simulink library "Transmission_Lib"  (R2025a)
settings: Solver=ode45  StartTime=0.0  StopTime=10.0  RelTol=1e-3  EnableMultiTasking=on
undefined symbols (not defined in the file): DCT_Param
libraries: fl_lib x45, nesl_utility x25, sdl_lib x18
(part 1 of 2)
Description:
  | Copyright 2014-2025 The MathWorks, Inc.
settings Model: Creator=smiller  LastModifiedBy=smiller
settings SolverCC: AlgebraicLoopSolver=TrustRegion
settings DataIOCC: SaveFormat=Array  SignalLoggingSaveFormat=ModelDataLogs  ReturnWorkspaceOutputs=off
settings OptimizationCC: ReuseModelBlockBuffer=off  ExpressionDepthLimit=2147483647.0  LifeSpan=inf
settings DebuggingCC: UnderspecifiedInitializationDetection=Classic  MergeDetectMultiDrivingBlocksExec=none  SolverPrmCheckMsg=warning  FcnCallInpInsideContextMsg=warning  UnconnectedInputMsg=warning  UnconnectedOutputMsg=warning  UnconnectedLineMsg=warning  AllowSymbolicDim=off  StateNameClashWarn=warning  PregeneratedLibrarySubsystemCodeDiagnostic=none  SFUnexpectedBacktrackingDiag=warning  SFNoUnconditionalDefaultTransitionDiag=warning  SFExecutionAtInitializationDiag=none  ArithmeticOperatorsInVariantConditions=warning
settings HardwareCC: ProdBitPerPointer=32.0  ProdBitPerSizeT=32.0  ProdBitPerPtrDiffT=32.0  ProdLargestAtomicFloat=None  ProdIntDivRoundTo=Undefined  ProdEndianess=Unspecified  ProdWordSize=32.0  ProdHWDeviceType=32-bit Generic
settings ModelReferenceCC: EnableRefExpFcnMdlSchedulingChecks=on  PropagateSignalLabelsOutOfModel=off
settings SFSimCC: SimUseLocalCustomCode=off  CustomCodeUndefinedFunction=UseInterfaceOnly
settings RTWCC: RTWUseLocalCustomCode=off  GPUComputeCapability=3.5  DLArmComputeVersion=19.05
settings CodeAppCC: StateflowObjectComments=on
settings GRTTargetCC: TargetLangStandard=C89/C90 (ANSI)  CombineOutputUpdateFcns=off  GRTInterface=on
settings ConfigComp: CovMetricSettings=dw  CovSaveCumulativeToWorkspaceVar=on  CovSaveSingleToWorkspaceVar=on  CovExternalEMLEnable=off  CovSFcnEnable=off

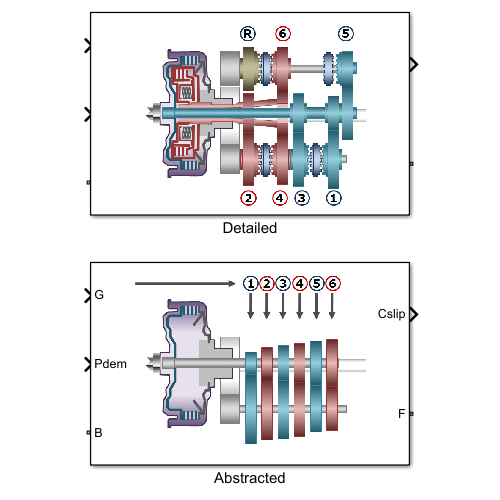
[thumbnail: Simulink's stored preview of the top-level diagram]
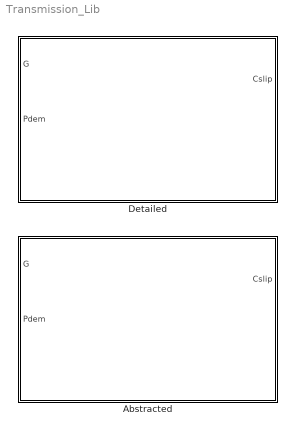
== system Transmission_Lib ==
  Abstracted : Subsystem
      mask Display: image(imread('DCT_Transmission_Abstracted_IMAGE2.jpg'));
  Detailed : Subsystem
      mask Display: image(imread('DCT_Transmission_IMAGE2.jpg'));

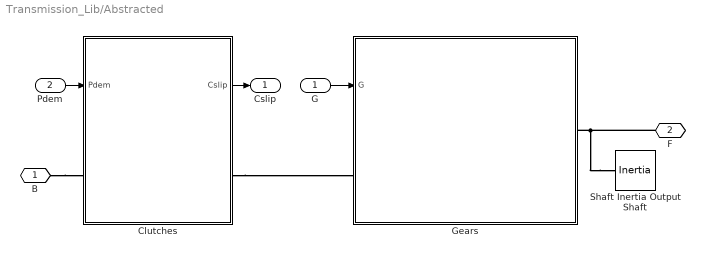
== system Transmission_Lib/Abstracted ==
  G : Inport
  Pdem : Inport  Port=2
  Clutches : Subsystem
      mask Display: image(imread('DCT_Clutches_Abstracted_IMAGE.jpg'));
  Gears : Subsystem
      mask Display: image(imread('DCT_Gears_Abstracted_IMAGE.jpg'));
  Shaft Inertia Output Shaft : fl_lib/Mechanical/Rotational Elements/Inertia  inertia=DCT_Param.Transmission.Shaft_Inertia_Output kg*m^2  num_ports=foundation.enum.numPorts2.one  w_specify=on  w_priority=High  w=DCT_Param.Transmission.Shaft_Velocity_Output rad/s  w_nominal_specify=off  w_nominal_value=1  w_nominal_unit=rad/s  t_specify=off  t_priority=High  t=0 N*m  t_nominal_specify=off  t_nominal_value=1  t_nominal_unit=N*m
  B : PMIOPort  Side=Left
  F : PMIOPort  Port=2  Side=Right
  Cslip : Outport  VectorParamsAs1DForOutWhenUnconnected=off
  wires:
  G/1 -> Gears/1(G)
  Clutches/1(Cslip) -> Cslip/1
  Pdem/1 -> Clutches/1(Pdem)
  connections:
  Shaft Inertia Output Shaft/LConn1 -- F/RConn1 -- Gears/RConn1
  Clutches/RConn1 -- Gears/LConn1
  B/RConn1 -- Clutches/LConn1

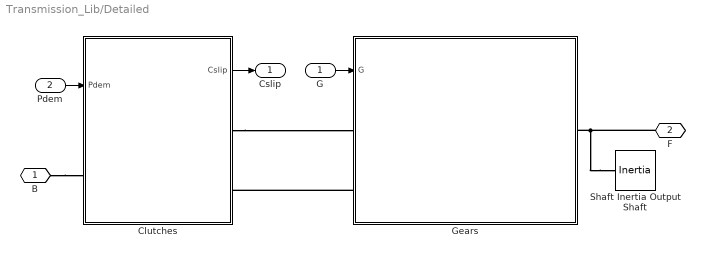
== system Transmission_Lib/Detailed ==
  G : Inport
  Pdem : Inport  Port=2
  Clutches : Subsystem
      mask Display:
      | image(imread('DCT_Clutches_IMAGE.jpg'));
      | port_label('input',1,'Pdem')
      | port_label('output',1,'Cslip')
      | port_label('LConn',1,'ICE')
      | port_label('RConn',1,'Odd')
      | port_label('RConn',2,'Even')
  Gears : Subsystem
      mask Display:
      | image(imread('DCT_Gears_IMAGE.jpg'));
      | port_label('input',1,'G')
      | port_label('LConn',1,'Odd')
      | port_label('LConn',2,'Even')
      | port_label('RConn',1,'F')
  Shaft Inertia Output Shaft : fl_lib/Mechanical/Rotational Elements/Inertia  inertia=DCT_Param.Transmission.Shaft_Inertia_Output kg*m^2  num_ports=foundation.enum.numPorts2.one  w_specify=on  w_priority=High  w=DCT_Param.Transmission.Shaft_Velocity_Output rad/s  w_nominal_specify=off  w_nominal_value=1  w_nominal_unit=rad/s  t_specify=off  t_priority=High  t=0 N*m  t_nominal_specify=off  t_nominal_value=1  t_nominal_unit=N*m
  B : PMIOPort  Side=Left
  F : PMIOPort  Port=2  Side=Right
  Cslip : Outport  VectorParamsAs1DForOutWhenUnconnected=off
  wires:
  G/1 -> Gears/1(G)
  Clutches/1(Cslip) -> Cslip/1
  Pdem/1 -> Clutches/1(Pdem)
  connections:
  Gears/LConn2 -- Clutches/RConn2
  Shaft Inertia Output Shaft/LConn1 -- F/RConn1 -- Gears/RConn1
  Clutches/RConn1 -- Gears/LConn1
  B/RConn1 -- Clutches/LConn1

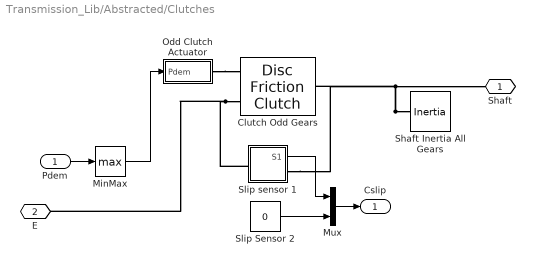
== system Transmission_Lib/Abstracted/Clutches ==
  Pdem : Inport
  Clutch Odd Gears : sdl_lib/Clutches/Disc Friction Clutch  geometry_model=1  r_eff=DCT_Param.Clutch.Torque_Radius mm  d_o=150 mm  d_i=100 mm  nS=DCT_Param.Clutch.Num_Friction_Surfaces  piston_area=DCT_Param.Clutch.Engagement_Piston_Area m^2  unidirectional=0  friction_model=1  mu_w_vector=[ 0 0.1 0.2 0.3 0.4 0.5 1 2 5 10 100 1000 ] rad/s  temperature_TLU=[280.0, 300.0, 320.0] K  mu_static=DCT_Param.Clutch.Static_Friction_Coeff  mu_static_vector=[0.4, 0.38, 0.36]  mu_coulomb=DCT_Param.Clutch.Kinetic_Friction_Coeff  mu_coulomb_vector=[ 0.29 0.28 0.26 0.22 0.21 0.2 0.2 0.19 0.19 0.19 0.19 0.19 ]  mu_coulomb_temp_vector=[0.3, 0.28, 0.25]  mu_coulomb_matrix=[0.34, 0.32, 0.3; 0.3, 0.28, 0.25; 0.25, 0.2, 0.15]  mu_interp_method=1  mu_extrap_method=1  d_f=DCT_Param.Clutch.Derating_Factor  w_tol=DCT_Param.Clutch.Clutch_Velocity_Tolerance rad/s  pressure_min=DCT_Param.Clutch.Threshold_Pressure Pa  mu_visc=DCT_Param.Clutch.Drag_Torque_Coeff N*m/(rad/s)  initial_state_locked=0  thermal_mass=25 kJ/K  T_init=300 K
      settings: InternalSimscapePortConfiguration="{\"Bottom\":[],\"Left\":[{\"id\":\"P\",\"label\":\"P\",\"type\":\"input\"},{\"id\":\"B\",\"label\":\"B\",\"type\":\"foundation.mechanical.rotational.rotational\"}],\"Right\":[{\"id\":\"F\",\"label\":\"F\",\"type\":\"foundation.mechanical.rotational.rotational\"}],\"Top\":[]}"
  MinMax : MinMax  Function=max
  Mux : Mux  Inputs=2
  Odd Clutch Actuator : Subsystem
  Shaft Inertia All Gears : fl_lib/Mechanical/Rotational Elements/Inertia  inertia=DCT_Param.Transmission.Shaft_Inertia_Odd kg*m^2  num_ports=foundation.enum.numPorts2.one  w_specify=on  w_priority=High  w=DCT_Param.Transmission.Shaft_Velocity_Odd rad/s  w_nominal_specify=off  w_nominal_value=1  w_nominal_unit=rad/s  t_specify=off  t_priority=High  t=0 N*m  t_nominal_specify=off  t_nominal_value=1  t_nominal_unit=N*m
  Slip Sensor 2 : Constant  Value=0
  Slip sensor 1 : Subsystem
  Shaft : PMIOPort  Side=Right
  E : PMIOPort  Port=2  Side=Left
  Cslip : Outport  VectorParamsAs1DForOutWhenUnconnected=off
  wires:
  Slip Sensor 2/1 -> Mux/2
  MinMax/1 -> Odd Clutch Actuator/1(Pdem)
  Pdem/1 -> MinMax/1
  Mux/1 -> Cslip/1
  Slip sensor 1/1(S1) -> Mux/1
  connections:
  Shaft Inertia All Gears/LConn1 -- Shaft/RConn1 -- Clutch Odd Gears/RConn1 -- Slip sensor 1/RConn1
  Odd Clutch Actuator/RConn1 -- Clutch Odd Gears/LConn1
  Clutch Odd Gears/LConn2 -- Slip sensor 1/LConn1 -- E/RConn1

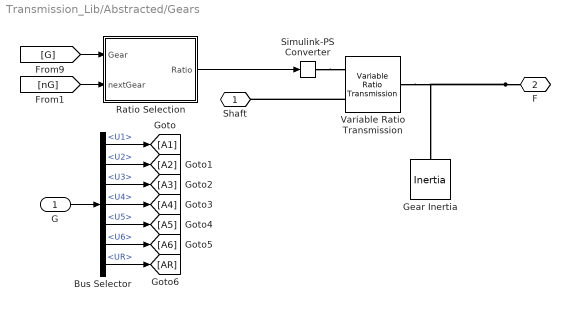
== system Transmission_Lib/Abstracted/Gears ==
  G : Inport
  Bus Selector : BusSelector  OutputSignals=U1,U2,U3,U4,U5,U6,UR
  Gear Inertia : fl_lib/Mechanical/Rotational Elements/Inertia  inertia=DCT_Param.Transmission.Gear_Inertia kg*m^2  num_ports=foundation.enum.numPorts2.one  w_specify=on  w_priority=High  w=0 rad/s  w_nominal_specify=off  w_nominal_value=1  w_nominal_unit=rad/s  t_specify=off  t_priority=High  t=0 N*m  t_nominal_specify=off  t_nominal_value=1  t_nominal_unit=N*m
  Ratio Selection : Subsystem
  Simulink-PS Converter : nesl_utility/Simulink-PS Converter  PhysicalDomain=network_engine_domain  SubClassName=ps_input  LeftPortType=input  RightPortType=output  PseudoPeriodic=off  Frequencies=[]  NoiseDistribution=none  NoiseParameters=[]  Unit=1  AffineConversion=off  FilteringAndDerivatives=zero  SimscapeFilterOrder=1  InputFilterTimeConstant=0.005  UdotUserProvided=0
  Variable Ratio Transmission : sdl_lib/Couplings & Drives/Variable Ratio Transmission  rotation_direction=3-2*(2)  kp=DCT_Param.Transmission.Abstract.Compliance N*m/rad  kv=DCT_Param.Transmission.Abstract.Damping N*m/(rad/s)  initial_torque=0 N*m  ratio_thr=0.01  losses_model=(1)-1  efficiency=0.85  pwr_thr=0.001 W  mu_visc=[ 0 0 ] N*m/(rad/s)
      settings: InternalSimscapePortConfiguration="{\"Bottom\":[],\"Left\":[{\"id\":\"ratio\",\"label\":\"r\",\"type\":\"input\"},{\"id\":\"B\",\"label\":\"B\",\"type\":\"foundation.mechanical.rotational.rotational\"}],\"Right\":[{\"id\":\"F\",\"label\":\"F\",\"type\":\"foundation.mechanical.rotational.rotational\"}],\"Top\":[]}"
  Shaft : PMIOPort  Side=Left
  F : PMIOPort  Port=2  Side=Right
  wires:
  [G] -> Ratio Selection/1(Gear)
  Ratio Selection/1(Ratio) -> Simulink-PS Converter/1
  Bus Selector/7 -> [AR]  "<UR>"
  Bus Selector/6 -> [A6]  "<U6>"
  Bus Selector/5 -> [A5]  "<U5>"
  Bus Selector/4 -> [A4]  "<U4>"
  Bus Selector/3 -> [A3]  "<U3>"
  Bus Selector/2 -> [A2]  "<U2>"
  Bus Selector/1 -> [A1]  "<U1>"
  G/1 -> Bus Selector/1
  [nG] -> Ratio Selection/2(nextGear)
  connections:
  Simulink-PS Converter/RConn1 -- Variable Ratio Transmission/LConn1
  F/RConn1 -- Gear Inertia/LConn1 -- Variable Ratio Transmission/RConn1
  Variable Ratio Transmission/LConn2 -- Shaft/RConn1

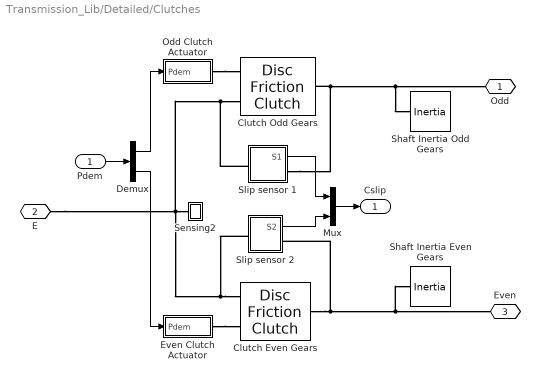
== system Transmission_Lib/Detailed/Clutches ==
  Pdem : Inport
  Clutch Even Gears : sdl_lib/Clutches/Disc Friction Clutch  Tag=CustomStyle  geometry_model=1  r_eff=DCT_Param.Clutch.Torque_Radius mm  d_o=150 mm  d_i=100 mm  nS=DCT_Param.Clutch.Num_Friction_Surfaces  piston_area=DCT_Param.Clutch.Engagement_Piston_Area m^2  unidirectional=0  friction_model=1  mu_w_vector=[ 0 0.1 0.2 0.3 0.4 0.5 1 2 5 10 100 1000 ] rad/s  temperature_TLU=[280.0, 300.0, 320.0] K  mu_static=DCT_Param.Clutch.Static_Friction_Coeff  mu_static_vector=[0.4, 0.38, 0.36]  mu_coulomb=DCT_Param.Clutch.Kinetic_Friction_Coeff  mu_coulomb_vector=[ 0.29 0.28 0.26 0.22 0.21 0.2 0.2 0.19 0.19 0.19 0.19 0.19 ]  mu_coulomb_temp_vector=[0.3, 0.28, 0.25]  mu_coulomb_matrix=[0.34, 0.32, 0.3; 0.3, 0.28, 0.25; 0.25, 0.2, 0.15]  mu_interp_method=1  mu_extrap_method=1  d_f=DCT_Param.Clutch.Derating_Factor  w_tol=DCT_Param.Clutch.Clutch_Velocity_Tolerance rad/s  pressure_min=DCT_Param.Clutch.Threshold_Pressure Pa  mu_visc=DCT_Param.Clutch.Drag_Torque_Coeff N*m/(rad/s)  initial_state_locked=0  thermal_mass=25 kJ/K  T_init=300 K
      settings: InternalSimscapePortConfiguration="{\"Bottom\":[],\"Left\":[{\"id\":\"P\",\"label\":\"P\",\"type\":\"input\"},{\"id\":\"B\",\"label\":\"B\",\"type\":\"foundation.mechanical.rotational.rotational\"}],\"Right\":[{\"id\":\"F\",\"label\":\"F\",\"type\":\"foundation.mechanical.rotational.rotational\"}],\"Top\":[]}"
  Clutch Odd Gears : sdl_lib/Clutches/Disc Friction Clutch  Tag=CustomStyle  geometry_model=1  r_eff=DCT_Param.Clutch.Torque_Radius mm  d_o=150 mm  d_i=100 mm  nS=DCT_Param.Clutch.Num_Friction_Surfaces  piston_area=DCT_Param.Clutch.Engagement_Piston_Area m^2  unidirectional=0  friction_model=1  mu_w_vector=[ 0 0.1 0.2 0.3 0.4 0.5 1 2 5 10 100 1000 ] rad/s  temperature_TLU=[280.0, 300.0, 320.0] K  mu_static=DCT_Param.Clutch.Static_Friction_Coeff  mu_static_vector=[0.4, 0.38, 0.36]  mu_coulomb=DCT_Param.Clutch.Kinetic_Friction_Coeff  mu_coulomb_vector=[ 0.29 0.28 0.26 0.22 0.21 0.2 0.2 0.19 0.19 0.19 0.19 0.19 ]  mu_coulomb_temp_vector=[0.3, 0.28, 0.25]  mu_coulomb_matrix=[0.34, 0.32, 0.3; 0.3, 0.28, 0.25; 0.25, 0.2, 0.15]  mu_interp_method=1  mu_extrap_method=1  d_f=DCT_Param.Clutch.Derating_Factor  w_tol=DCT_Param.Clutch.Clutch_Velocity_Tolerance rad/s  pressure_min=DCT_Param.Clutch.Threshold_Pressure Pa  mu_visc=DCT_Param.Clutch.Drag_Torque_Coeff N*m/(rad/s)  initial_state_locked=0  thermal_mass=25 kJ/K  T_init=300 K
      settings: InternalSimscapePortConfiguration="{\"Bottom\":[],\"Left\":[{\"id\":\"P\",\"label\":\"P\",\"type\":\"input\"},{\"id\":\"B\",\"label\":\"B\",\"type\":\"foundation.mechanical.rotational.rotational\"}],\"Right\":[{\"id\":\"F\",\"label\":\"F\",\"type\":\"foundation.mechanical.rotational.rotational\"}],\"Top\":[]}"
  Demux : Demux  Outputs=2
  Even Clutch Actuator : Subsystem
  Mux : Mux  Inputs=2
  Odd Clutch Actuator : Subsystem
  Sensing2 : Subsystem
  Shaft Inertia Even Gears : fl_lib/Mechanical/Rotational Elements/Inertia  inertia=DCT_Param.Transmission.Shaft_Inertia_Even kg*m^2  num_ports=foundation.enum.numPorts2.one  w_specify=on  w_priority=High  w=DCT_Param.Transmission.Shaft_Velocity_Even rad/s  w_nominal_specify=off  w_nominal_value=1  w_nominal_unit=rad/s  t_specify=off  t_priority=High  t=0 N*m  t_nominal_specify=off  t_nominal_value=1  t_nominal_unit=N*m
  Shaft Inertia Odd Gears : fl_lib/Mechanical/Rotational Elements/Inertia  inertia=DCT_Param.Transmission.Shaft_Inertia_Odd kg*m^2  num_ports=foundation.enum.numPorts2.one  w_specify=on  w_priority=High  w=DCT_Param.Transmission.Shaft_Velocity_Odd rad/s  w_nominal_specify=off  w_nominal_value=1  w_nominal_unit=rad/s  t_specify=off  t_priority=High  t=0 N*m  t_nominal_specify=off  t_nominal_value=1  t_nominal_unit=N*m
  Slip sensor 1 : Subsystem
  Slip sensor 2 : Subsystem
  Odd : PMIOPort  Side=Right
  E : PMIOPort  Port=2  Side=Left
  Even : PMIOPort  Port=3  Side=Right
  Cslip : Outport  VectorParamsAs1DForOutWhenUnconnected=off
  wires:
  Demux/2 -> Even Clutch Actuator/1(Pdem)
  Demux/1 -> Odd Clutch Actuator/1(Pdem)
  Pdem/1 -> Demux/1
  Mux/1 -> Cslip/1
  Slip sensor 2/1(S2) -> Mux/2
  Slip sensor 1/1(S1) -> Mux/1
  connections:
  Shaft Inertia Odd Gears/LConn1 -- Odd/RConn1 -- Clutch Odd Gears/RConn1 -- Slip sensor 1/RConn1
  Odd Clutch Actuator/RConn1 -- Clutch Odd Gears/LConn1
  Shaft Inertia Even Gears/LConn1 -- Even/RConn1 -- Clutch Even Gears/RConn1 -- Slip sensor 2/RConn1
  Clutch Even Gears/LConn2 -- Slip sensor 2/LConn1 -- E/RConn1 -- Sensing2/LConn1 -- Clutch Odd Gears/LConn2 -- Slip sensor 1/LConn1
  Even Clutch Actuator/RConn1 -- Clutch Even Gears/LConn1

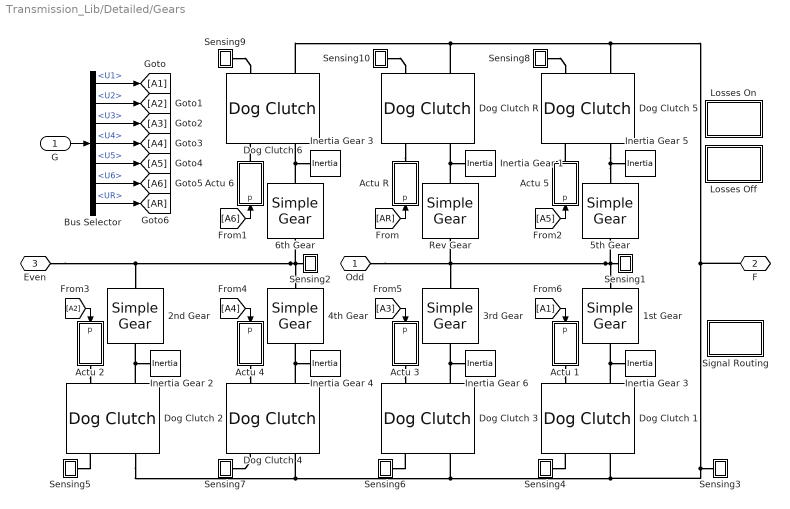
== system Transmission_Lib/Detailed/Gears ==
  G : Inport
  1st Gear : sdl_lib/Gears/Simple Gear  Tag=CustomStyle  ratio=DCT_Param.Transmission.Ratios(1)  rotation_direction=3-2*(2)  friction_model=1  T_noload=0.1 N*m  T_nom=5 N*m  efficiency_nom=0.8  efficiency=DCT_Param.Transmission.Gear_Efficiency  temperature_TLU=[ 280 300 320 ] K  load_TLU=[ 1 5 10 ] N*m  efficiency_TLU=[ 0.95 0.9 0.85 ]  efficiency_TLU2=[ 0.85 0.8 0.75; 0.95 0.9 0.85; 0.85 0.8 0.7 ]  w_thr=DCT_Param.Transmission.Gear_Ang_Vel_Thr rad/s  pwr_thr=0.001 W  enable_backlash=false  hardstop_model=simscape.enum.hardstop.smooth  backlash_distance=1e-3 mm  r_base=0.1 m  transition=1e-4 mm  backlash_stiffness=1e7 N/m  backlash_damping=1e6 N*s/m  coeff_rest=0  v_tol=0.001 m/s  f_tol=0 N  mu_visc=[0 0] N*m/(rad/s)  thermal_mass=50 J/K  temperature_specify=off  temperature_priority=High  temperature=300 K  temperature_nominal_specify=off  temperature_nominal_value=1  temperature_nominal_unit=K  x_backlash_specify=off  x_backlash_priority=None  x_backlash=0 mm  x_backlash_nominal_specify=off  x_backlash_nominal_value=1  x_backlash_nominal_unit=mm  f_hardstop_specify=off  f_hardstop_priority=None  f_hardstop=0 N  f_hardstop_nominal_specify=off  f_hardstop_nominal_value=1  f_hardstop_nominal_unit=N  v_backlash_specify=off  v_backlash_priority=None  v_backlash=0 m/s  v_backlash_nominal_specify=off  v_backlash_nominal_value=1  v_backlash_nominal_unit=m/s
  2nd Gear : sdl_lib/Gears/Simple Gear  Tag=CustomStyle  ratio=DCT_Param.Transmission.Ratios(2)  rotation_direction=3-2*(2)  friction_model=1  T_noload=0.1 N*m  T_nom=5 N*m  efficiency_nom=0.8  efficiency=DCT_Param.Transmission.Gear_Efficiency  temperature_TLU=[ 280 300 320 ] K  load_TLU=[ 1 5 10 ] N*m  efficiency_TLU=[ 0.95 0.9 0.85 ]  efficiency_TLU2=[ 0.85 0.8 0.75; 0.95 0.9 0.85; 0.85 0.8 0.7 ]  w_thr=DCT_Param.Transmission.Gear_Ang_Vel_Thr rad/s  pwr_thr=0.001 W  enable_backlash=false  hardstop_model=simscape.enum.hardstop.smooth  backlash_distance=1e-3 mm  r_base=0.1 m  transition=1e-4 mm  backlash_stiffness=1e7 N/m  backlash_damping=1e6 N*s/m  coeff_rest=0  v_tol=0.001 m/s  f_tol=0 N  mu_visc=[0 0] N*m/(rad/s)  thermal_mass=50 J/K  temperature_specify=off  temperature_priority=High  temperature=300 K  temperature_nominal_specify=off  temperature_nominal_value=1  temperature_nominal_unit=K  x_backlash_specify=off  x_backlash_priority=None  x_backlash=0 mm  x_backlash_nominal_specify=off  x_backlash_nominal_value=1  x_backlash_nominal_unit=mm  f_hardstop_specify=off  f_hardstop_priority=None  f_hardstop=0 N  f_hardstop_nominal_specify=off  f_hardstop_nominal_value=1  f_hardstop_nominal_unit=N  v_backlash_specify=off  v_backlash_priority=None  v_backlash=0 m/s  v_backlash_nominal_specify=off  v_backlash_nominal_value=1  v_backlash_nominal_unit=m/s
  3rd Gear : sdl_lib/Gears/Simple Gear  Tag=CustomStyle  ratio=DCT_Param.Transmission.Ratios(3)  rotation_direction=3-2*(2)  friction_model=1  T_noload=0.1 N*m  T_nom=5 N*m  efficiency_nom=0.8  efficiency=DCT_Param.Transmission.Gear_Efficiency  temperature_TLU=[ 280 300 320 ] K  load_TLU=[ 1 5 10 ] N*m  efficiency_TLU=[ 0.95 0.9 0.85 ]  efficiency_TLU2=[ 0.85 0.8 0.75; 0.95 0.9 0.85; 0.85 0.8 0.7 ]  w_thr=DCT_Param.Transmission.Gear_Ang_Vel_Thr rad/s  pwr_thr=0.001 W  enable_backlash=false  hardstop_model=simscape.enum.hardstop.smooth  backlash_distance=1e-3 mm  r_base=0.1 m  transition=1e-4 mm  backlash_stiffness=1e7 N/m  backlash_damping=1e6 N*s/m  coeff_rest=0  v_tol=0.001 m/s  f_tol=0 N  mu_visc=[0 0] N*m/(rad/s)  thermal_mass=50 J/K  temperature_specify=off  temperature_priority=High  temperature=300 K  temperature_nominal_specify=off  temperature_nominal_value=1  temperature_nominal_unit=K  x_backlash_specify=off  x_backlash_priority=None  x_backlash=0 mm  x_backlash_nominal_specify=off  x_backlash_nominal_value=1  x_backlash_nominal_unit=mm  f_hardstop_specify=off  f_hardstop_priority=None  f_hardstop=0 N  f_hardstop_nominal_specify=off  f_hardstop_nominal_value=1  f_hardstop_nominal_unit=N  v_backlash_specify=off  v_backlash_priority=None  v_backlash=0 m/s  v_backlash_nominal_specify=off  v_backlash_nominal_value=1  v_backlash_nominal_unit=m/s
  4th Gear : sdl_lib/Gears/Simple Gear  Tag=CustomStyle  ratio=DCT_Param.Transmission.Ratios(4)  rotation_direction=3-2*(2)  friction_model=1  T_noload=0.1 N*m  T_nom=5 N*m  efficiency_nom=0.8  efficiency=DCT_Param.Transmission.Gear_Efficiency  temperature_TLU=[ 280 300 320 ] K  load_TLU=[ 1 5 10 ] N*m  efficiency_TLU=[ 0.95 0.9 0.85 ]  efficiency_TLU2=[ 0.85 0.8 0.75; 0.95 0.9 0.85; 0.85 0.8 0.7 ]  w_thr=DCT_Param.Transmission.Gear_Ang_Vel_Thr rad/s  pwr_thr=0.001 W  enable_backlash=false  hardstop_model=simscape.enum.hardstop.smooth  backlash_distance=1e-3 mm  r_base=0.1 m  transition=1e-4 mm  backlash_stiffness=1e7 N/m  backlash_damping=1e6 N*s/m  coeff_rest=0  v_tol=0.001 m/s  f_tol=0 N  mu_visc=[0 0] N*m/(rad/s)  thermal_mass=50 J/K  temperature_specify=off  temperature_priority=High  temperature=300 K  temperature_nominal_specify=off  temperature_nominal_value=1  temperature_nominal_unit=K  x_backlash_specify=off  x_backlash_priority=None  x_backlash=0 mm  x_backlash_nominal_specify=off  x_backlash_nominal_value=1  x_backlash_nominal_unit=mm  f_hardstop_specify=off  f_hardstop_priority=None  f_hardstop=0 N  f_hardstop_nominal_specify=off  f_hardstop_nominal_value=1  f_hardstop_nominal_unit=N  v_backlash_specify=off  v_backlash_priority=None  v_backlash=0 m/s  v_backlash_nominal_specify=off  v_backlash_nominal_value=1  v_backlash_nominal_unit=m/s
  5th Gear : sdl_lib/Gears/Simple Gear  Tag=CustomStyle  ratio=DCT_Param.Transmission.Ratios(5)  rotation_direction=3-2*(2)  friction_model=1  T_noload=0.1 N*m  T_nom=5 N*m  efficiency_nom=0.8  efficiency=DCT_Param.Transmission.Gear_Efficiency  temperature_TLU=[ 280 300 320 ] K  load_TLU=[ 1 5 10 ] N*m  efficiency_TLU=[ 0.95 0.9 0.85 ]  efficiency_TLU2=[ 0.85 0.8 0.75; 0.95 0.9 0.85; 0.85 0.8 0.7 ]  w_thr=DCT_Param.Transmission.Gear_Ang_Vel_Thr rad/s  pwr_thr=0.001 W  enable_backlash=false  hardstop_model=simscape.enum.hardstop.smooth  backlash_distance=1e-3 mm  r_base=0.1 m  transition=1e-4 mm  backlash_stiffness=1e7 N/m  backlash_damping=1e6 N*s/m  coeff_rest=0  v_tol=0.001 m/s  f_tol=0 N  mu_visc=[0 0] N*m/(rad/s)  thermal_mass=50 J/K  temperature_specify=off  temperature_priority=High  temperature=300 K  temperature_nominal_specify=off  temperature_nominal_value=1  temperature_nominal_unit=K  x_backlash_specify=off  x_backlash_priority=None  x_backlash=0 mm  x_backlash_nominal_specify=off  x_backlash_nominal_value=1  x_backlash_nominal_unit=mm  f_hardstop_specify=off  f_hardstop_priority=None  f_hardstop=0 N  f_hardstop_nominal_specify=off  f_hardstop_nominal_value=1  f_hardstop_nominal_unit=N  v_backlash_specify=off  v_backlash_priority=None  v_backlash=0 m/s  v_backlash_nominal_specify=off  v_backlash_nominal_value=1  v_backlash_nominal_unit=m/s
  6th Gear : sdl_lib/Gears/Simple Gear  Tag=CustomStyle  ratio=DCT_Param.Transmission.Ratios(6)  rotation_direction=3-2*(2)  friction_model=1  T_noload=0.1 N*m  T_nom=5 N*m  efficiency_nom=0.8  efficiency=DCT_Param.Transmission.Gear_Efficiency  temperature_TLU=[ 280 300 320 ] K  load_TLU=[ 1 5 10 ] N*m  efficiency_TLU=[ 0.95 0.9 0.85 ]  efficiency_TLU2=[ 0.85 0.8 0.75; 0.95 0.9 0.85; 0.85 0.8 0.7 ]  w_thr=DCT_Param.Transmission.Gear_Ang_Vel_Thr rad/s  pwr_thr=0.001 W  enable_backlash=false  hardstop_model=simscape.enum.hardstop.smooth  backlash_distance=1e-3 mm  r_base=0.1 m  transition=1e-4 mm  backlash_stiffness=1e7 N/m  backlash_damping=1e6 N*s/m  coeff_rest=0  v_tol=0.001 m/s  f_tol=0 N  mu_visc=[0 0] N*m/(rad/s)  thermal_mass=50 J/K  temperature_specify=off  temperature_priority=High  temperature=300 K  temperature_nominal_specify=off  temperature_nominal_value=1  temperature_nominal_unit=K  x_backlash_specify=off  x_backlash_priority=None  x_backlash=0 mm  x_backlash_nominal_specify=off  x_backlash_nominal_value=1  x_backlash_nominal_unit=mm  f_hardstop_specify=off  f_hardstop_priority=None  f_hardstop=0 N  f_hardstop_nominal_specify=off  f_hardstop_nominal_value=1  f_hardstop_nominal_unit=N  v_backlash_specify=off  v_backlash_priority=None  v_backlash=0 m/s  v_backlash_nominal_specify=off  v_backlash_nominal_value=1  v_backlash_nominal_unit=m/s
  Actu 1 : Subsystem
  Actu 2 : Subsystem
  Actu 3 : Subsystem
  Actu 4 : Subsystem
  Actu 5 : Subsystem
  Actu 6 : Subsystem
  Actu R : Subsystem
  Bus Selector : BusSelector  OutputSignals=U1,U2,U3,U4,U5,U6,UR
  Dog Clutch 1 : sdl_lib/Clutches/Dog Clutch  Tag=CustomStyle  model=1  w_threshold=5 rpm  thermal_port=simscape.enum.thermaleffects.omit  radius=DCT_Param.Dog_Clutch.Teeth_Mean_Radius mm  max_torque=DCT_Param.Dog_Clutch.Max_Torque N*m  n_teeth=6  temperature_TLU=[280.0, 300.0, 320.0] K  max_torque_vector=[1000.0, 1050.0, 1000.0] N*m  interp_method=1  extrap_method=1  clutch_backlash=10 deg  clutch_stiffness=1e+7 N*m/rad  clutch_damping=2 N*m/(rad/s)  shift_linkage_twomode=sdl.enum.shift_linkage_twomode.logic  shift_linkage=sdl.enum.shift_linkage.conserving  tooth_height=DCT_Param.Dog_Clutch.Tooth_Height mm  ring_hub_gap=DCT_Param.Dog_Clutch.Ring_Hub_Clearance mm  back_stop=1  transl_stiffness=DCT_Param.Dog_Clutch.Ring_Stop_Stiffness N/m  transl_damping=DCT_Param.Dog_Clutch.Ring_Stop_Damping N/(m/s)  visc_fric_transl=DCT_Param.Dog_Clutch.Shift_Linkage_Damping N/(m/s)  engaged_fric_transl=100 N*s/m  disengaged_fric_transl=50 N*s/m  v_tol=0.1 m/s  f_tol=0.001 N  fric_coeff=0.05  direction=3-2*(1)  engagement_velocity=DCT_Param.Dog_Clutch.Max_Engage_Velocity rad/s  engagement_overlap=DCT_Param.Dog_Clutch.Tooth_Engage_Overlap mm  engagement_block_stiffness=10e6 N/m  engagement_block_damping=300 N*s/m  initial_state_engaged=1  init_pos=DCT_Param.Dog_Clutch.Tooth_Height+DCT_Param.Dog_Clutch.Ring_Hub_Clearance mm  init_rel_angle=0 deg  thermal_mass=25 kJ/K  T_init=300 K
      settings: InternalSimscapePortConfiguration="{\"Bottom\":[],\"Left\":[{\"id\":\"S\",\"label\":\"S\",\"type\":\"foundation.mechanical.translational.translational\"},{\"id\":\"R\",\"label\":\"R\",\"type\":\"foundation.mechanical.rotational.rotational\"}],\"Right\":[{\"id\":\"X\",\"label\":\"X\",\"type\":\"output\"},{\"id\":\"H\",\"label\":\"H\",\"type\":\"foundation.mechanical.rotational.rotational\"}],\"Top\":[]}"
  Dog Clutch {2..6} (5 alike) : sdl_lib/Clutches/Dog Clutch  Tag=CustomStyle  model=1  w_threshold=5 rpm  thermal_port=simscape.enum.thermaleffects.omit  radius=DCT_Param.Dog_Clutch.Teeth_Mean_Radius mm  max_torque=DCT_Param.Dog_Clutch.Max_Torque N*m  n_teeth=6  temperature_TLU=[280.0, 300.0, 320.0] K  max_torque_vector=[1000.0, 1050.0, 1000.0] N*m  interp_method=1  extrap_method=1  clutch_backlash=10 deg  clutch_stiffness=1e+7 N*m/rad  clutch_damping=2 N*m/(rad/s)  shift_linkage_twomode=sdl.enum.shift_linkage_twomode.logic  shift_linkage=sdl.enum.shift_linkage.conserving  tooth_height=DCT_Param.Dog_Clutch.Tooth_Height mm  ring_hub_gap=DCT_Param.Dog_Clutch.Ring_Hub_Clearance mm  back_stop=1  transl_stiffness=DCT_Param.Dog_Clutch.Ring_Stop_Stiffness N/m  transl_damping=DCT_Param.Dog_Clutch.Ring_Stop_Damping N/(m/s)  visc_fric_transl=DCT_Param.Dog_Clutch.Shift_Linkage_Damping N/(m/s)  engaged_fric_transl=100 N*s/m  disengaged_fric_transl=50 N*s/m  v_tol=0.1 m/s  f_tol=0.001 N  fric_coeff=0.05  direction=3-2*(1)  engagement_velocity=DCT_Param.Dog_Clutch.Max_Engage_Velocity rad/s  engagement_overlap=DCT_Param.Dog_Clutch.Tooth_Engage_Overlap mm  engagement_block_stiffness=10e6 N/m  engagement_block_damping=300 N*s/m  initial_state_engaged=0  init_pos=0 mm  init_rel_angle=0 deg  thermal_mass=25 kJ/K  T_init=300 K
      settings: InternalSimscapePortConfiguration="{\"Bottom\":[],\"Left\":[{\"id\":\"S\",\"label\":\"S\",\"type\":\"foundation.mechanical.translational.translational\"},{\"id\":\"R\",\"label\":\"R\",\"type\":\"foundation.mechanical.rotational.rotational\"}],\"Right\":[{\"id\":\"X\",\"label\":\"X\",\"type\":\"output\"},{\"id\":\"H\",\"label\":\"H\",\"type\":\"foundation.mechanical.rotational.rotational\"}],\"Top\":[]}"
  Dog Clutch R : sdl_lib/Clutches/Dog Clutch  Tag=CustomStyle  model=1  w_threshold=5 rpm  thermal_port=simscape.enum.thermaleffects.omit  radius=DCT_Param.Dog_Clutch.Teeth_Mean_Radius mm  max_torque=DCT_Param.Dog_Clutch.Max_Torque N*m  n_teeth=6  temperature_TLU=[280.0, 300.0, 320.0] K  max_torque_vector=[1000.0, 1050.0, 1000.0] N*m  interp_method=1  extrap_method=1  clutch_backlash=10 deg  clutch_stiffness=1e+7 N*m/rad  clutch_damping=2 N*m/(rad/s)  shift_linkage_twomode=sdl.enum.shift_linkage_twomode.logic  shift_linkage=sdl.enum.shift_linkage.conserving  tooth_height=DCT_Param.Dog_Clutch.Tooth_Height mm  ring_hub_gap=DCT_Param.Dog_Clutch.Ring_Hub_Clearance mm  back_stop=1  transl_stiffness=DCT_Param.Dog_Clutch.Ring_Stop_Stiffness N/m  transl_damping=DCT_Param.Dog_Clutch.Ring_Stop_Damping N/(m/s)  visc_fric_transl=DCT_Param.Dog_Clutch.Shift_Linkage_Damping N/(m/s)  engaged_fric_transl=100 N*s/m  disengaged_fric_transl=50 N*s/m  v_tol=0.1 m/s  f_tol=0.001 N  fric_coeff=0.05  direction=3-2*(1)  engagement_velocity=DCT_Param.Dog_Clutch.Max_Engage_Velocity rad/s  engagement_overlap=DCT_Param.Dog_Clutch.Tooth_Engage_Overlap mm  engagement_block_stiffness=10e6 N/m  engagement_block_damping=300 N*s/m  initial_state_engaged=0  init_pos=0 mm  init_rel_angle=0 deg  thermal_mass=25 kJ/K  T_init=300 K
      settings: InternalSimscapePortConfiguration="{\"Bottom\":[],\"Left\":[{\"id\":\"S\",\"label\":\"S\",\"type\":\"foundation.mechanical.translational.translational\"},{\"id\":\"R\",\"label\":\"R\",\"type\":\"foundation.mechanical.rotational.rotational\"}],\"Right\":[{\"id\":\"X\",\"label\":\"X\",\"type\":\"output\"},{\"id\":\"H\",\"label\":\"H\",\"type\":\"foundation.mechanical.rotational.rotational\"}],\"Top\":[]}"
  Inertia Gear {1..6} (6 alike) : fl_lib/Mechanical/Rotational Elements/Inertia  inertia=DCT_Param.Transmission.Gear_Inertia kg*m^2  num_ports=foundation.enum.numPorts2.one  w_specify=on  w_priority=High  w=DCT_Param.Transmission.Gear_Initial_Velocity rad/s  w_nominal_specify=off  w_nominal_value=1  w_nominal_unit=rad/s  t_specify=off  t_priority=High  t=0 N*m  t_nominal_specify=off  t_nominal_value=1  t_nominal_unit=N*m
  "Inertia Gear 3 " : fl_lib/Mechanical/Rotational Elements/Inertia  inertia=DCT_Param.Transmission.Gear_Inertia kg*m^2  num_ports=foundation.enum.numPorts2.one  w_specify=on  w_priority=High  w=DCT_Param.Transmission.Gear_Initial_Velocity rad/s  w_nominal_specify=off  w_nominal_value=1  w_nominal_unit=rad/s  t_specify=off  t_priority=High  t=0 N*m  t_nominal_specify=off  t_nominal_value=1  t_nominal_unit=N*m
  Losses Off : Subsystem
      settings: OpenFcn=|
      | gearblk_h = find_system(gcs,'MatchFilter',@Simulink.match.allVariants,'ClassName','simple_gear');
      | for i = 1:length(gearblk_h)
      | set_param(gearblk_h{i},'friction_model','1'); end
      mask Display: disp('Losses\nOff');
  Losses On : Subsystem
      settings: OpenFcn=|
      | gearblk_h = find_system(gcs,'MatchFilter',@Simulink.match.allVariants,'ClassName','simple_gear');
      | for i = 1:length(gearblk_h)
      | set_param(gearblk_h{i},'friction_model','2'); end;
      mask Display: disp('Losses\nOn');
  Rev Gear : sdl_lib/Gears/Simple Gear  Tag=CustomStyle  ratio=DCT_Param.Transmission.Ratios(1)  rotation_direction=3-2*(1)  friction_model=1  T_noload=0.1 N*m  T_nom=5 N*m  efficiency_nom=0.8  efficiency=DCT_Param.Transmission.Gear_Efficiency  temperature_TLU=[ 280 300 320 ] K  load_TLU=[ 1 5 10 ] N*m  efficiency_TLU=[ 0.95 0.9 0.85 ]  efficiency_TLU2=[ 0.85 0.8 0.75; 0.95 0.9 0.85; 0.85 0.8 0.7 ]  w_thr=DCT_Param.Transmission.Gear_Ang_Vel_Thr rad/s  pwr_thr=0.001 W  enable_backlash=false  hardstop_model=simscape.enum.hardstop.smooth  backlash_distance=1e-3 mm  r_base=0.1 m  transition=1e-4 mm  backlash_stiffness=1e7 N/m  backlash_damping=1e6 N*s/m  coeff_rest=0  v_tol=0.001 m/s  f_tol=0 N  mu_visc=[0 0] N*m/(rad/s)  thermal_mass=50 J/K  temperature_specify=off  temperature_priority=High  temperature=300 K  temperature_nominal_specify=off  temperature_nominal_value=1  temperature_nominal_unit=K  x_backlash_specify=off  x_backlash_priority=None  x_backlash=0 mm  x_backlash_nominal_specify=off  x_backlash_nominal_value=1  x_backlash_nominal_unit=mm  f_hardstop_specify=off  f_hardstop_priority=None  f_hardstop=0 N  f_hardstop_nominal_specify=off  f_hardstop_nominal_value=1  f_hardstop_nominal_unit=N  v_backlash_specify=off  v_backlash_priority=None  v_backlash=0 m/s  v_backlash_nominal_specify=off  v_backlash_nominal_value=1  v_backlash_nominal_unit=m/s
  Sensing1 : Subsystem
  Sensing10 : Subsystem
  Sensing2 : Subsystem
  Sensing3 : Subsystem
  Sensing4 : Subsystem
  Sensing5 : Subsystem
  Sensing6 : Subsystem
  Sensing7 : Subsystem
  Sensing8 : Subsystem
  Sensing9 : Subsystem
  Signal Routing : Subsystem
  Odd : PMIOPort  Side=Left
  F : PMIOPort  Port=2  Side=Right
  Even : PMIOPort  Port=3  Side=Left
  wires:
  Bus Selector/7 -> [AR]  "<UR>"
  [AR] -> Actu R/1(p)
  [A1] -> Actu 1/1(p)
  Bus Selector/6 -> [A6]  "<U6>"
  Bus Selector/5 -> [A5]  "<U5>"
  Bus Selector/4 -> [A4]  "<U4>"
  Bus Selector/3 -> [A3]  "<U3>"
  Bus Selector/2 -> [A2]  "<U2>"
  Bus Selector/1 -> [A1]  "<U1>"
  [A3] -> Actu 3/1(p)
  [A4] -> Actu 4/1(p)
  [A2] -> Actu 2/1(p)
  [A5] -> Actu 5/1(p)
  [A6] -> Actu 6/1(p)
  G/1 -> Bus Selector/1
  connections:
  Sensing10/LConn1 -- Dog Clutch R/RConn1
  Sensing9/LConn1 -- Dog Clutch 6/RConn1
  Sensing8/LConn1 -- Dog Clutch 5/RConn1
  Sensing7/LConn1 -- Dog Clutch 4/RConn1
  Sensing6/LConn1 -- Dog Clutch 3/RConn1
  Sensing5/LConn1 -- Dog Clutch 2/RConn1
  Sensing4/LConn1 -- Dog Clutch 1/RConn1
  Dog Clutch R/LConn1 -- Actu R/RConn1
  Dog Clutch R/LConn2 -- Rev Gear/RConn1 -- Inertia Gear 1/LConn1
  Sensing3/LConn1 -- Dog Clutch 1/RConn2 -- Dog Clutch 3/RConn2 -- Dog Clutch 4/RConn2 -- Dog Clutch 2/RConn2 -- F/RConn1 -- Dog Clutch 5/RConn2 -- Dog Clutch R/RConn2 -- Dog Clutch 6/RConn2
  5th Gear/LConn1 -- Rev Gear/LConn1 -- 3rd Gear/LConn1 -- Odd/RConn1 -- Sensing1/LConn1 -- 1st Gear/LConn1
  6th Gear/LConn1 -- 2nd Gear/LConn1 -- Even/RConn1 -- Sensing2/LConn1 -- 4th Gear/LConn1
  Actu 1/RConn1 -- Dog Clutch 1/LConn1
  Dog Clutch 1/LConn2 -- 1st Gear/RConn1 -- Inertia Gear 3/LConn1
  Actu 4/RConn1 -- Dog Clutch 4/LConn1
  Actu 5/RConn1 -- Dog Clutch 5/LConn1
  Actu 6/RConn1 -- Dog Clutch 6/LConn1
  Actu 2/RConn1 -- Dog Clutch 2/LConn1
  Actu 3/RConn1 -- Dog Clutch 3/LConn1
  3rd Gear/RConn1 -- Dog Clutch 3/LConn2 -- Inertia Gear 6/LConn1
  4th Gear/RConn1 -- Dog Clutch 4/LConn2 -- Inertia Gear 4/LConn1
  2nd Gear/RConn1 -- Dog Clutch 2/LConn2 -- Inertia Gear 2/LConn1
  5th Gear/RConn1 -- Dog Clutch 5/LConn2 -- Inertia Gear 5/LConn1
  Dog Clutch 6/LConn2 -- 6th Gear/RConn1 -- "Inertia Gear 3 "/LConn1

== system Transmission_Lib/Abstracted/Clutches/Odd Clutch Actuator ==
  Pdem : Inport
  Pressure controller time constant : TransferFcn  Denominator=[0.02 1]
  Simulink-PS Converter : nesl_utility/Simulink-PS Converter  PhysicalDomain=network_engine_domain  SubClassName=ps_input  LeftPortType=input  RightPortType=output  PseudoPeriodic=off  Frequencies=[]  NoiseDistribution=none  NoiseParameters=[]  Unit=Pa  AffineConversion=off  FilteringAndDerivatives=zero  SimscapeFilterOrder=1  InputFilterTimeConstant=0.005  UdotUserProvided=0
  P : PMIOPort  Side=Right
  wires:
  Pdem/1 -> Pressure controller time constant/1
  Pressure controller time constant/1 -> Simulink-PS Converter/1
  connections:
  P/RConn1 -- Simulink-PS Converter/RConn1

== system Transmission_Lib/Abstracted/Clutches/Slip sensor 1 ==
  Ideal Rotational Motion Sensor : fl_lib/Mechanical/Mechanical Sensors/Ideal Rotational Motion Sensor  reference=foundation.enum.MeasurementReference.difference  acceleration_port=false  velocity_port=true  position_port=true  wrap_angle=simscape.enum.onoff.off  offset=0 rad
  PS-Simulink Converter3 : nesl_utility/PS-Simulink Converter  PhysicalDomain=network_engine_domain  SubClassName=ps_output  LeftPortType=input  RightPortType=output  PseudoPeriodic=off  Frequencies=[]  VectorFormat=1-D array  Unit=rpm  AffineConversion=off
  Zero-Order Hold : ZeroOrderHold  SampleTime=0.01
  F : PMIOPort  Side=Right
  B : PMIOPort  Port=2  Side=Left
  S1 : Outport  VectorParamsAs1DForOutWhenUnconnected=off
  wires:
  Zero-Order Hold/1 -> S1/1
  PS-Simulink Converter3/1 -> Zero-Order Hold/1
  connections:
  B/RConn1 -- Ideal Rotational Motion Sensor/LConn1
  F/RConn1 -- Ideal Rotational Motion Sensor/RConn1
  Ideal Rotational Motion Sensor/RConn2 -- PS-Simulink Converter3/LConn1

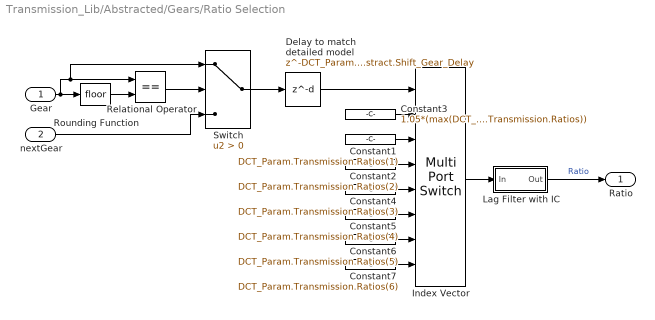
== system Transmission_Lib/Abstracted/Gears/Ratio Selection ==
  Gear : Inport
  nextGear : Inport  Port=2
  Constant1 : Constant  Value=DCT_Param.Transmission.Ratios(1)
  Constant2 : Constant  Value=DCT_Param.Transmission.Ratios(2)
  Constant3 : Constant  Value=1.05*(max(DCT_Param.Transmission.Ratios))
  Constant4 : Constant  Value=DCT_Param.Transmission.Ratios(3)
  Constant5 : Constant  Value=DCT_Param.Transmission.Ratios(4)
  Constant6 : Constant  Value=DCT_Param.Transmission.Ratios(5)
  Constant7 : Constant  Value=DCT_Param.Transmission.Ratios(6)
  Delay to match detailed model : Delay  DelayLength=DCT_Param.Transmission.Abstract.Shift_Gear_Delay  InitialCondition=1  SampleTime=0.01
  Index Vector : MultiPortSwitch  DataPortOrder=Zero-based contiguous  Inputs=7  zeroidx=on  SaturateOnIntegerOverflow=off  InputSameDT=off
  Lag Filter with IC : Subsystem  mask(First-order lag supporting vector signals){b=DCT_Param.Transmission.Abstract.Ratio_Time_Const, x_initial=DCT_Param.Transmission.Ratios(1)}
      mask prompts: b "Filter time constant"; x_initial "Initial output"
      mask help: Models a lag of the form 1/(b*s+1) where s is the Laplace operator.
  Relational Operator : RelationalOperator  Operator===  OutDataTypeStr=boolean  InputSameDT=off
  Rounding Function : Rounding
  Switch : Switch  Criteria=u2 > Threshold  SaturateOnIntegerOverflow=off  InputSameDT=off
  Ratio : Outport  VectorParamsAs1DForOutWhenUnconnected=off
  wires:
  Index Vector/1 -> Lag Filter with IC/1(In)
  Constant7/1 -> Index Vector/8
  Constant6/1 -> Index Vector/7
  Constant5/1 -> Index Vector/6
  Constant4/1 -> Index Vector/5
  Constant2/1 -> Index Vector/4
  Constant1/1 -> Index Vector/3
  Constant3/1 -> Index Vector/2
  Gear/1 -> Rounding Function/1, Relational Operator/1, Switch/1
  Lag Filter with IC/1(Out) -> Ratio/1  "Ratio"
  Rounding Function/1 -> Relational Operator/2
  Relational Operator/1 -> Switch/2
  Switch/1 -> Delay to match detailed model/1
  nextGear/1 -> Switch/3
  Delay to match detailed model/1 -> Index Vector/1

== system Transmission_Lib/Detailed/Clutches/Even Clutch Actuator ==
  Pdem : Inport
  Pressure controller time constant : TransferFcn  Denominator=[0.02 1]
  Simulink-PS Converter1 : nesl_utility/Simulink-PS Converter  PhysicalDomain=network_engine_domain  SubClassName=ps_input  LeftPortType=input  RightPortType=output  PseudoPeriodic=off  Frequencies=[]  NoiseDistribution=none  NoiseParameters=[]  Unit=Pa  AffineConversion=off  FilteringAndDerivatives=zero  SimscapeFilterOrder=1  InputFilterTimeConstant=0.005  UdotUserProvided=0
  P : PMIOPort  Side=Right
  wires:
  Pdem/1 -> Pressure controller time constant/1
  Pressure controller time constant/1 -> Simulink-PS Converter1/1
  connections:
  P/RConn1 -- Simulink-PS Converter1/RConn1

== system Transmission_Lib/Detailed/Clutches/Odd Clutch Actuator ==
  Pdem : Inport
  Pressure controller time constant : TransferFcn  Denominator=[0.02 1]
  Simulink-PS Converter : nesl_utility/Simulink-PS Converter  PhysicalDomain=network_engine_domain  SubClassName=ps_input  LeftPortType=input  RightPortType=output  PseudoPeriodic=off  Frequencies=[]  NoiseDistribution=none  NoiseParameters=[]  Unit=Pa  AffineConversion=off  FilteringAndDerivatives=zero  SimscapeFilterOrder=1  InputFilterTimeConstant=0.005  UdotUserProvided=0
  P : PMIOPort  Side=Right
  wires:
  Pdem/1 -> Pressure controller time constant/1
  Pressure controller time constant/1 -> Simulink-PS Converter/1
  connections:
  P/RConn1 -- Simulink-PS Converter/RConn1

== system Transmission_Lib/Detailed/Clutches/Sensing2 ==
  Ideal Rotational Motion Sensor : fl_lib/Mechanical/Mechanical Sensors/Ideal Rotational Motion Sensor  reference=foundation.enum.MeasurementReference.difference  acceleration_port=false  velocity_port=true  position_port=true  wrap_angle=simscape.enum.onoff.off  offset=0 rad
  Integrator : Integrator
  Mechanical Rotational Reference : fl_lib/Mechanical/Rotational Elements/Mechanical Rotational Reference
  PS-Simulink Converter : nesl_utility/PS-Simulink Converter  PhysicalDomain=network_engine_domain  SubClassName=ps_output  LeftPortType=input  RightPortType=output  PseudoPeriodic=off  Frequencies=[]  VectorFormat=1-D array  Unit=1  AffineConversion=off
  S : PMIOPort  Side=Left
  tag scope: DCT_Inp_Engine_Sh_Ang=global
  wires:
  PS-Simulink Converter/1 -> Integrator/1
  Integrator/1 -> [DCT_Inp_Engine_Sh_Ang]
  connections:
  Mechanical Rotational Reference/LConn1 -- Ideal Rotational Motion Sensor/RConn1
  PS-Simulink Converter/LConn1 -- Ideal Rotational Motion Sensor/RConn3
  S/RConn1 -- Ideal Rotational Motion Sensor/LConn1

== system Transmission_Lib/Detailed/Clutches/Slip sensor 1 ==
  Ideal Rotational Motion Sensor : fl_lib/Mechanical/Mechanical Sensors/Ideal Rotational Motion Sensor  reference=foundation.enum.MeasurementReference.difference  acceleration_port=false  velocity_port=true  position_port=true  wrap_angle=simscape.enum.onoff.off  offset=0 rad
  PS-Simulink Converter3 : nesl_utility/PS-Simulink Converter  PhysicalDomain=network_engine_domain  SubClassName=ps_output  LeftPortType=input  RightPortType=output  PseudoPeriodic=off  Frequencies=[]  VectorFormat=1-D array  Unit=rpm  AffineConversion=off
  Sensing4 : Subsystem
  Zero-Order Hold : ZeroOrderHold  SampleTime=0.01
  F : PMIOPort  Side=Right
  B : PMIOPort  Port=2  Side=Left
  S1 : Outport  VectorParamsAs1DForOutWhenUnconnected=off
  wires:
  Zero-Order Hold/1 -> S1/1
  PS-Simulink Converter3/1 -> Sensing4/1(S), Zero-Order Hold/1
  connections:
  B/RConn1 -- Ideal Rotational Motion Sensor/LConn1
  F/RConn1 -- Ideal Rotational Motion Sensor/RConn1
  Ideal Rotational Motion Sensor/RConn2 -- PS-Simulink Converter3/LConn1

== system Transmission_Lib/Detailed/Clutches/Slip sensor 2 ==
  Ideal Rotational Motion Sensor : fl_lib/Mechanical/Mechanical Sensors/Ideal Rotational Motion Sensor  reference=foundation.enum.MeasurementReference.difference  acceleration_port=false  velocity_port=true  position_port=true  wrap_angle=simscape.enum.onoff.off  offset=0 rad
  PS-Simulink Converter3 : nesl_utility/PS-Simulink Converter  PhysicalDomain=network_engine_domain  SubClassName=ps_output  LeftPortType=input  RightPortType=output  PseudoPeriodic=off  Frequencies=[]  VectorFormat=1-D array  Unit=rpm  AffineConversion=off
  Sensing4 : Subsystem
  Zero-Order Hold : ZeroOrderHold  SampleTime=0.01
  F : PMIOPort  Side=Right
  B : PMIOPort  Port=2  Side=Left
  S2 : Outport  VectorParamsAs1DForOutWhenUnconnected=off
  wires:
  Zero-Order Hold/1 -> S2/1
  PS-Simulink Converter3/1 -> Sensing4/1(S), Zero-Order Hold/1
  connections:
  Ideal Rotational Motion Sensor/RConn2 -- PS-Simulink Converter3/LConn1
  F/RConn1 -- Ideal Rotational Motion Sensor/RConn1
  B/RConn1 -- Ideal Rotational Motion Sensor/LConn1

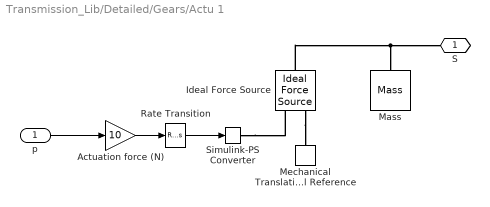
== system Transmission_Lib/Detailed/Gears/Actu 1 ==
  p : Inport
  Actuation force (N) : Gain  Gain=10  SaturateOnIntegerOverflow=on  OutDataTypeStr=Inherit: Same as input  ParamDataTypeStr=Inherit: Same as input
  Ideal Force Source : fl_lib/Mechanical/Mechanical Sources/Ideal Force Source
  Mass : fl_lib/Mechanical/Translational Elements/Mass  mass=0.5 kg  num_ports=foundation.enum.numPorts2.one  v_specify=on  v_priority=High  v=0 m/s  v_nominal_specify=off  v_nominal_value=1  v_nominal_unit=m/s  f_specify=off  f_priority=High  f=0 N  f_nominal_specify=off  f_nominal_value=1  f_nominal_unit=N
  Mechanical Translational Reference : fl_lib/Mechanical/Translational Elements/Mechanical Translational Reference
  Rate Transition : RateTransition
  Simulink-PS Converter : nesl_utility/Simulink-PS Converter  PhysicalDomain=network_engine_domain  SubClassName=ps_input  LeftPortType=input  RightPortType=output  PseudoPeriodic=off  Frequencies=[]  NoiseDistribution=none  NoiseParameters=[]  Unit=1  AffineConversion=off  FilteringAndDerivatives=zero  SimscapeFilterOrder=1  InputFilterTimeConstant=0.005  UdotUserProvided=0
  S : PMIOPort  Side=Right
  wires:
  p/1 -> Actuation force (N)/1
  Actuation force (N)/1 -> Rate Transition/1
  Rate Transition/1 -> Simulink-PS Converter/1
  connections:
  Ideal Force Source/RConn2 -- Mechanical Translational Reference/LConn1
  Ideal Force Source/LConn1 -- S/RConn1 -- Mass/LConn1
  Simulink-PS Converter/RConn1 -- Ideal Force Source/RConn1

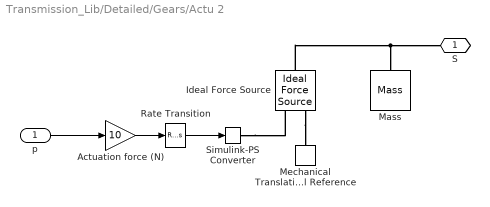
== system Transmission_Lib/Detailed/Gears/Actu 2 ==
  p : Inport
  Actuation force (N) : Gain  Gain=10  SaturateOnIntegerOverflow=on  OutDataTypeStr=Inherit: Same as input  ParamDataTypeStr=Inherit: Same as input
  Ideal Force Source : fl_lib/Mechanical/Mechanical Sources/Ideal Force Source
  Mass : fl_lib/Mechanical/Translational Elements/Mass  mass=0.5 kg  num_ports=foundation.enum.numPorts2.one  v_specify=on  v_priority=High  v=0 m/s  v_nominal_specify=off  v_nominal_value=1  v_nominal_unit=m/s  f_specify=off  f_priority=High  f=0 N  f_nominal_specify=off  f_nominal_value=1  f_nominal_unit=N
  Mechanical Translational Reference : fl_lib/Mechanical/Translational Elements/Mechanical Translational Reference
  Rate Transition : RateTransition
  Simulink-PS Converter : nesl_utility/Simulink-PS Converter  PhysicalDomain=network_engine_domain  SubClassName=ps_input  LeftPortType=input  RightPortType=output  PseudoPeriodic=off  Frequencies=[]  NoiseDistribution=none  NoiseParameters=[]  Unit=1  AffineConversion=off  FilteringAndDerivatives=zero  SimscapeFilterOrder=1  InputFilterTimeConstant=0.005  UdotUserProvided=0
  S : PMIOPort  Side=Right
  wires:
  p/1 -> Actuation force (N)/1
  Actuation force (N)/1 -> Rate Transition/1
  Rate Transition/1 -> Simulink-PS Converter/1
  connections:
  Ideal Force Source/RConn2 -- Mechanical Translational Reference/LConn1
  Ideal Force Source/LConn1 -- S/RConn1 -- Mass/LConn1
  Simulink-PS Converter/RConn1 -- Ideal Force Source/RConn1

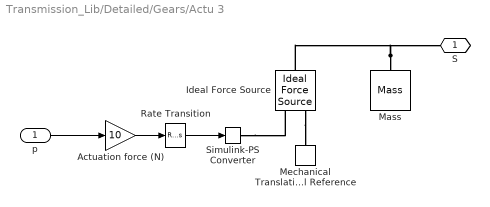
== system Transmission_Lib/Detailed/Gears/Actu 3 ==
  p : Inport
  Actuation force (N) : Gain  Gain=10  SaturateOnIntegerOverflow=on  OutDataTypeStr=Inherit: Same as input  ParamDataTypeStr=Inherit: Same as input
  Ideal Force Source : fl_lib/Mechanical/Mechanical Sources/Ideal Force Source
  Mass : fl_lib/Mechanical/Translational Elements/Mass  mass=0.5 kg  num_ports=foundation.enum.numPorts2.one  v_specify=on  v_priority=High  v=0 m/s  v_nominal_specify=off  v_nominal_value=1  v_nominal_unit=m/s  f_specify=off  f_priority=High  f=0 N  f_nominal_specify=off  f_nominal_value=1  f_nominal_unit=N
  Mechanical Translational Reference : fl_lib/Mechanical/Translational Elements/Mechanical Translational Reference
  Rate Transition : RateTransition
  Simulink-PS Converter : nesl_utility/Simulink-PS Converter  PhysicalDomain=network_engine_domain  SubClassName=ps_input  LeftPortType=input  RightPortType=output  PseudoPeriodic=off  Frequencies=[]  NoiseDistribution=none  NoiseParameters=[]  Unit=1  AffineConversion=off  FilteringAndDerivatives=zero  SimscapeFilterOrder=1  InputFilterTimeConstant=0.005  UdotUserProvided=0
  S : PMIOPort  Side=Right
  wires:
  Rate Transition/1 -> Simulink-PS Converter/1
  Actuation force (N)/1 -> Rate Transition/1
  p/1 -> Actuation force (N)/1
  connections:
  Simulink-PS Converter/RConn1 -- Ideal Force Source/RConn1
  Mass/LConn1 -- S/RConn1 -- Ideal Force Source/LConn1
  Ideal Force Source/RConn2 -- Mechanical Translational Reference/LConn1

== system Transmission_Lib/Detailed/Gears/Actu 4 ==
  p : Inport
  Actuation force (N) : Gain  Gain=10  SaturateOnIntegerOverflow=on  OutDataTypeStr=Inherit: Same as input  ParamDataTypeStr=Inherit: Same as input
  Ideal Force Source : fl_lib/Mechanical/Mechanical Sources/Ideal Force Source
  Mass : fl_lib/Mechanical/Translational Elements/Mass  mass=0.5 kg  num_ports=foundation.enum.numPorts2.one  v_specify=on  v_priority=High  v=0 m/s  v_nominal_specify=off  v_nominal_value=1  v_nominal_unit=m/s  f_specify=off  f_priority=High  f=0 N  f_nominal_specify=off  f_nominal_value=1  f_nominal_unit=N
  Mechanical Translational Reference : fl_lib/Mechanical/Translational Elements/Mechanical Translational Reference
  Rate Transition : RateTransition
  Simulink-PS Converter : nesl_utility/Simulink-PS Converter  PhysicalDomain=network_engine_domain  SubClassName=ps_input  LeftPortType=input  RightPortType=output  PseudoPeriodic=off  Frequencies=[]  NoiseDistribution=none  NoiseParameters=[]  Unit=1  AffineConversion=off  FilteringAndDerivatives=zero  SimscapeFilterOrder=1  InputFilterTimeConstant=0.005  UdotUserProvided=0
  S : PMIOPort  Side=Right
  wires:
  p/1 -> Actuation force (N)/1
  Actuation force (N)/1 -> Rate Transition/1
  Rate Transition/1 -> Simulink-PS Converter/1
  connections:
  Ideal Force Source/RConn2 -- Mechanical Translational Reference/LConn1
  Ideal Force Source/LConn1 -- S/RConn1 -- Mass/LConn1
  Simulink-PS Converter/RConn1 -- Ideal Force Source/RConn1

== system Transmission_Lib/Detailed/Gears/Actu 5 ==
  p : Inport
  Actuation force (N) : Gain  Gain=10  SaturateOnIntegerOverflow=on  OutDataTypeStr=Inherit: Same as input  ParamDataTypeStr=Inherit: Same as input
  Ideal Force Source : fl_lib/Mechanical/Mechanical Sources/Ideal Force Source
  Mass : fl_lib/Mechanical/Translational Elements/Mass  mass=0.5 kg  num_ports=foundation.enum.numPorts2.one  v_specify=on  v_priority=High  v=0 m/s  v_nominal_specify=off  v_nominal_value=1  v_nominal_unit=m/s  f_specify=off  f_priority=High  f=0 N  f_nominal_specify=off  f_nominal_value=1  f_nominal_unit=N
  Mechanical Translational Reference : fl_lib/Mechanical/Translational Elements/Mechanical Translational Reference
  Rate Transition : RateTransition
  Simulink-PS Converter : nesl_utility/Simulink-PS Converter  PhysicalDomain=network_engine_domain  SubClassName=ps_input  LeftPortType=input  RightPortType=output  PseudoPeriodic=off  Frequencies=[]  NoiseDistribution=none  NoiseParameters=[]  Unit=1  AffineConversion=off  FilteringAndDerivatives=zero  SimscapeFilterOrder=1  InputFilterTimeConstant=0.005  UdotUserProvided=0
  S : PMIOPort  Side=Right
  wires:
  p/1 -> Actuation force (N)/1
  Actuation force (N)/1 -> Rate Transition/1
  Rate Transition/1 -> Simulink-PS Converter/1
  connections:
  Ideal Force Source/RConn2 -- Mechanical Translational Reference/LConn1
  Ideal Force Source/LConn1 -- S/RConn1 -- Mass/LConn1
  Simulink-PS Converter/RConn1 -- Ideal Force Source/RConn1
